simulink model "peltier_lazo_P_lineal"  (R2026a)
settings: Solver=ode23t  StopTime=t_final  MaxStep=0.2  RelTol=1e-6  AbsTol=1e-8
values from neighbouring files (symbols this model uses):
  A = [-0.016283702978  0.0139822207014; 0.0172580552658  -0.0400425685209]    [parametros.mat]    (also in peltier_modelo.m = [ -(1/p.RCA + p.K + p.alpha*I)/p.CC,  p.K/p.CC)
  B = [-0.291897811742 0.532459698891]    [parametros.mat]    (also in peltier_modelo.m = [ -bC/p.CC ;  bH/p.CH ])
  denG = [1 0.0563262714989 0.000410735354666]    [parametros.mat]    (also in peltier_modelo.m = denG/denG(1))
  I0 = 1.19014918446    [parametros.mat]    (also in parametros_control.mat; peltier_modelo.m = fzero(@(I) [1 0]*equilibrio(I, p) - Tb_obj, [0, 2]); sensibilidad_P.m = fzero(@(i) temperatura_fria(i,p)-(10+273.15),[0 2]); sensibilidad_compensado.m = fzero(@(i) temperatura_fria(i,p)-(10+273.15),[0 2]))
  Imax = 2.0    (= 2)    [editar_ensayos.m]    (also in parametros_ensayos.mat)
  Imin = 0    [editar_ensayos.m]    (also in parametros_ensayos.mat)
  instante_ref = t_ref    [configurar.m]    (also in sensibilidad_P.m; sensibilidad_compensado.m; simular_P.m)
  Kp = Kp_base    [configurar.m]    (also in diseno_compensador.m = Kp_lista(i); sensibilidad_P.m; sensibilidad_compensado.m; simular_P.m = Kp_lista(k))
  numG = [-0.291897811742 -0.00424336910329]    [parametros.mat]    (also in peltier_modelo.m = numG/denG(1))
  p =     [parametros.mat]    (also in sensibilidad_P.m = p_nom; sensibilidad_compensado.m = p_nom; simular_P.m = p_nom)
  tau_corriente = 0.01    [editar_ensayos.m]    (also in parametros_ensayos.mat)
  Tc0 = 278.15    [parametros.mat]    (also in peltier_modelo.m = x0(1); sensibilidad_P.m = xe(1); sensibilidad_compensado.m = xe(1); simular_P.m = Tc0_nom)
  Tc_init = Tc0    [configurar.m]    (also in sensibilidad_P.m; sensibilidad_compensado.m; simular_P.m = p.Tamb)
  Th0 = 304.101077495    [parametros.mat]    (also in peltier_modelo.m = x0(2); sensibilidad_P.m = xe(2); sensibilidad_compensado.m = xe(2); simular_P.m = Th0_nom)
  Th_init = Th0    [configurar.m]    (also in sensibilidad_P.m; sensibilidad_compensado.m; simular_P.m = p.Tamb)
Description:
  | GR09 - P. e=Tb_medida-ref; mando=sat(I0+Kp*e,0,2); tau*dI/dt=mando-I.
settings Model: Creator=charl  LastModifiedBy=charl
settings DebuggingCC: AlgebraicLoopMsg=error

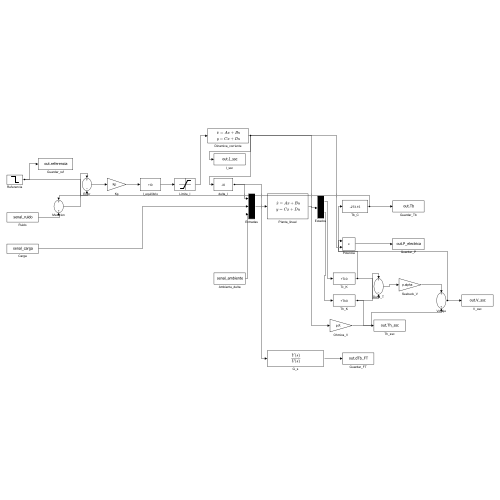
[thumbnail: Simulink's stored preview of the top-level diagram]
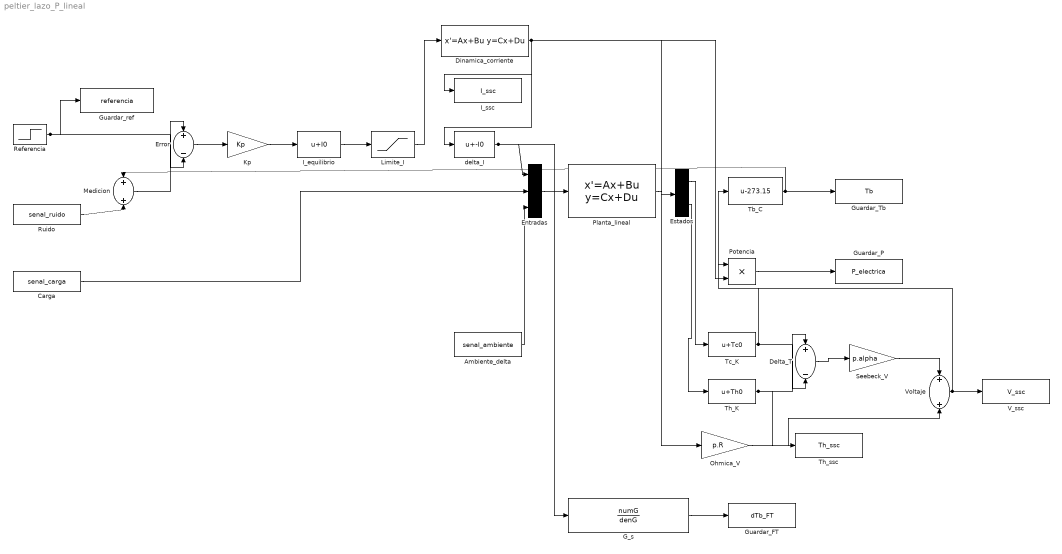
== system peltier_lazo_P_lineal ==
  Ambiente_delta : FromWorkspace  VariableName=senal_ambiente  Interpolate=off  OutputAfterFinalValue=Holding final value
  Carga : FromWorkspace  VariableName=senal_carga  Interpolate=off  OutputAfterFinalValue=Holding final value
  Delta_T : Sum  Inputs=+-
  Dinamica_corriente : StateSpace  A=-1/tau_corriente  B=1/tau_corriente  D=0  InitialCondition=I0
  Entradas : Mux  Inputs=3
  Error : Sum  Inputs=+-
  Estados : Demux  Outputs=2
  G_s : TransferFcn  Numerator=numG  Denominator=denG
  Guardar_FT : ToWorkspace  VariableName=dTb_FT  SaveFormat=Timeseries  SampleTime=-1
  Guardar_P : ToWorkspace  VariableName=P_electrica  SaveFormat=Timeseries  SampleTime=-1
  Guardar_Tb : ToWorkspace  VariableName=Tb  SaveFormat=Timeseries  SampleTime=-1
  Guardar_ref : ToWorkspace  VariableName=referencia  SaveFormat=Timeseries  SampleTime=-1
  I_equilibrio : Bias  Bias=I0  SaturateOnIntegerOverflow=off
  I_ssc : ToWorkspace  VariableName=I_ssc  SaveFormat=Timeseries  SampleTime=-1
  Kp : Gain  Gain=Kp
  Limite_I : Saturate  UpperLimit=Imax  LowerLimit=Imin
  Medicion : Sum
  Ohmica_V : Gain  Gain=p.R
  Planta_lineal : StateSpace  A=A  B=[B [1/p.CC;0] [1/(p.CC*p.RCA);1/(p.CH*p.RHA)]]  C=eye(2)  D=zeros(2,3)  InitialCondition=[Tc_init-Tc0;Th_init-Th0]
  Potencia : Product
  Referencia : Step  Time=instante_ref  InitialValue=r_antes  FinalValue=r_despues  SampleTime=0
  Ruido : FromWorkspace  VariableName=senal_ruido  Interpolate=off  OutputAfterFinalValue=Holding final value
  Seebeck_V : Gain  Gain=p.alpha
  Tb_C : Bias  Bias=-273.15  SaturateOnIntegerOverflow=off
  Tc_K : Bias  Bias=Tc0  SaturateOnIntegerOverflow=off
  Th_K : Bias  Bias=Th0  SaturateOnIntegerOverflow=off
  Th_ssc : ToWorkspace  VariableName=Th_ssc  SaveFormat=Timeseries  SampleTime=-1
  V_ssc : ToWorkspace  VariableName=V_ssc  SaveFormat=Timeseries  SampleTime=-1
  Voltaje : Sum
  delta_I : Bias  Bias=-I0  SaturateOnIntegerOverflow=off
  wires:
  Ruido/1 -> Medicion/2
  Tb_C/1 -> Medicion/1, Guardar_Tb/1
  Medicion/1 -> Error/1
  Referencia/1 -> Error/2, Guardar_ref/1
  Error/1 -> Kp/1
  Kp/1 -> I_equilibrio/1
  I_equilibrio/1 -> Limite_I/1
  Limite_I/1 -> Dinamica_corriente/1
  Potencia/1 -> Guardar_P/1
  Dinamica_corriente/1 -> delta_I/1, I_ssc/1, Ohmica_V/1, Potencia/2
  delta_I/1 -> Entradas/1, G_s/1
  Carga/1 -> Entradas/2
  Ambiente_delta/1 -> Entradas/3
  Entradas/1 -> Planta_lineal/1
  Planta_lineal/1 -> Estados/1
  Estados/1 -> Tc_K/1
  Estados/2 -> Th_K/1
  Tc_K/1 -> Tb_C/1, Delta_T/2
  Th_K/1 -> Delta_T/1, Th_ssc/1
  Delta_T/1 -> Seebeck_V/1
  Seebeck_V/1 -> Voltaje/1
  Ohmica_V/1 -> Voltaje/2
  Voltaje/1 -> V_ssc/1, Potencia/1
  G_s/1 -> Guardar_FT/1
